simulink model "WarehouseFleetSim"  (R2024b)
settings: Solver=ode4  StartTime=0.0  StopTime=inf  FixedStep=0.02  RelTol=1e-3
StopFcn:
  | try, fleetVisionStep('close'); catch, end; try, phase3('stopped'); catch, end
model workspace (MAT data in the model file):
  HomePose1 = [-20 7.3 0]
  HomePose2 = [-20 3.6 0]
  HomePose3 = [-20 11 0]
  HomePose4 = [-24.5 3.6 0]
  HomePose5 = [-24.5 7.3 0]
  HomePose6 = [-24.5 11 0]
  Zero = 0
  gen3 : robotics.RigidBodyTree (value not decoded)
  qStow = [0; 0; 0.261799387799; 3.14159265359; -2.26892802759; 0; 0.959931088597; 1.57079632679]
undefined symbols (not defined in the file or in its folder): Actor, setupFleetScene, Sim3dSensor, World
libraries: sim3dlib x128, sim3dcameralib x7, robotmobilelib x6, robotsim3dlib x6
(part 1 of 4)
settings Model: Creator=ssuga  LastModifiedBy=ssuga
settings DataIOCC: ReturnWorkspaceOutputs=off

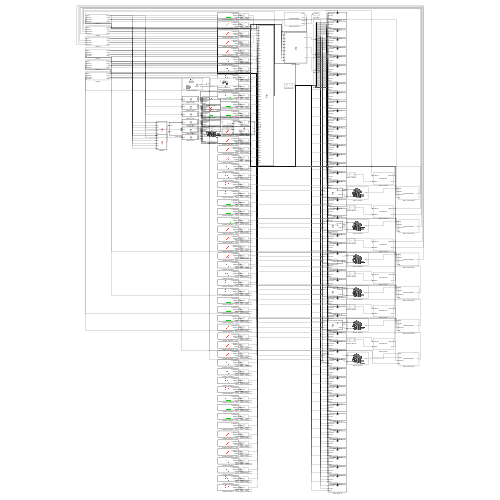
[thumbnail: Simulink's stored preview of the top-level diagram]
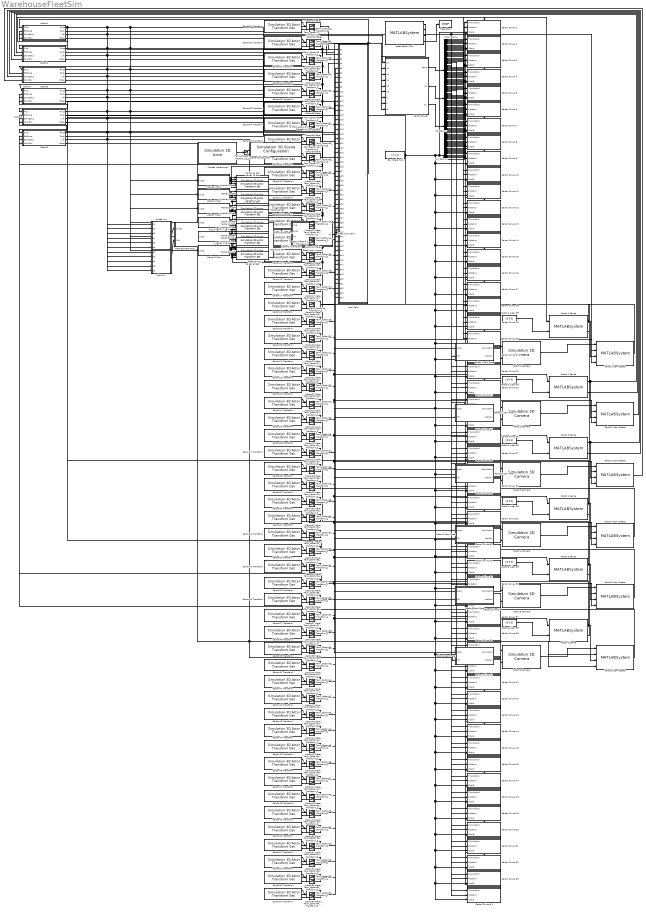
== system WarehouseFleetSim ==
  Box Scale Hold : Constant  Value=[1 1 1]  VectorParams1D=off  OutDataTypeStr=double
  Carton Driver 1 : Subsystem  TreatAsAtomicUnit=on
  Carton Driver 10 : Subsystem  TreatAsAtomicUnit=on
  Carton Driver 11 : Subsystem  TreatAsAtomicUnit=on
  Carton Driver 12 : Subsystem  TreatAsAtomicUnit=on
  Carton Driver 13 : Subsystem  TreatAsAtomicUnit=on
  Carton Driver 14 : Subsystem  TreatAsAtomicUnit=on
  Carton Driver 15 : Subsystem  TreatAsAtomicUnit=on
  Carton Driver 16 : Subsystem  TreatAsAtomicUnit=on
  Carton Driver 17 : Subsystem  TreatAsAtomicUnit=on
  Carton Driver 18 : Subsystem  TreatAsAtomicUnit=on
  Carton Driver 19 : Subsystem  TreatAsAtomicUnit=on
  Carton Driver 2 : Subsystem  TreatAsAtomicUnit=on
  Carton Driver 20 : Subsystem  TreatAsAtomicUnit=on
  Carton Driver 21 : Subsystem  TreatAsAtomicUnit=on
  Carton Driver 22 : Subsystem  TreatAsAtomicUnit=on
  Carton Driver 23 : Subsystem  TreatAsAtomicUnit=on
  Carton Driver 24 : Subsystem  TreatAsAtomicUnit=on
  Carton Driver 25 : Subsystem  TreatAsAtomicUnit=on
  Carton Driver 26 : Subsystem  TreatAsAtomicUnit=on
  Carton Driver 27 : Subsystem  TreatAsAtomicUnit=on
  Carton Driver 28 : Subsystem  TreatAsAtomicUnit=on
  Carton Driver 29 : Subsystem  TreatAsAtomicUnit=on
  Carton Driver 3 : Subsystem  TreatAsAtomicUnit=on
  Carton Driver 30 : Subsystem  TreatAsAtomicUnit=on
  Carton Driver 31 : Subsystem  TreatAsAtomicUnit=on
  Carton Driver 32 : Subsystem  TreatAsAtomicUnit=on
  Carton Driver 33 : Subsystem  TreatAsAtomicUnit=on
  Carton Driver 34 : Subsystem  TreatAsAtomicUnit=on
  Carton Driver 35 : Subsystem  TreatAsAtomicUnit=on
  Carton Driver 36 : Subsystem  TreatAsAtomicUnit=on
  Carton Driver 37 : Subsystem  TreatAsAtomicUnit=on
  Carton Driver 38 : Subsystem  TreatAsAtomicUnit=on
  Carton Driver 39 : Subsystem  TreatAsAtomicUnit=on
  Carton Driver 4 : Subsystem  TreatAsAtomicUnit=on
  Carton Driver 40 : Subsystem  TreatAsAtomicUnit=on
  Carton Driver 41 : Subsystem  TreatAsAtomicUnit=on
  Carton Driver 42 : Subsystem  TreatAsAtomicUnit=on
  Carton Driver 43 : Subsystem  TreatAsAtomicUnit=on
  Carton Driver 44 : Subsystem  TreatAsAtomicUnit=on
  Carton Driver 45 : Subsystem  TreatAsAtomicUnit=on
  Carton Driver 46 : Subsystem  TreatAsAtomicUnit=on
  Carton Driver 47 : Subsystem  TreatAsAtomicUnit=on
  Carton Driver 48 : Subsystem  TreatAsAtomicUnit=on
  Carton Driver 49 : Subsystem  TreatAsAtomicUnit=on
  Carton Driver 5 : Subsystem  TreatAsAtomicUnit=on
  Carton Driver 50 : Subsystem  TreatAsAtomicUnit=on
  Carton Driver 51 : Subsystem  TreatAsAtomicUnit=on
  Carton Driver 52 : Subsystem  TreatAsAtomicUnit=on
  Carton Driver 53 : Subsystem  TreatAsAtomicUnit=on
  Carton Driver 54 : Subsystem  TreatAsAtomicUnit=on
  Carton Driver 6 : Subsystem  TreatAsAtomicUnit=on
  Carton Driver 7 : Subsystem  TreatAsAtomicUnit=on
  Carton Driver 8 : Subsystem  TreatAsAtomicUnit=on
  Carton Driver 9 : Subsystem  TreatAsAtomicUnit=on
  Carton Router : MATLAB Function  TreatAsAtomicUnit=on
  Carton01 Delay : UnitDelay  InitialCondition=[-23.225 -38 1.43]  SampleTime=0.02  HasFrameUpgradeWarning=on
  Carton01 Transform : sim3dlib/Simulation 3D Actor Transform Get  Priority=1  ActorTag=Carton01  NumberOfParts=1  CustNumOfParts=3  Ts=-1  aMode=aMode
  Carton02 Delay : UnitDelay  InitialCondition=[-9.775 -51.4642857142857 0.53]  SampleTime=0.02  HasFrameUpgradeWarning=on
  Carton02 Transform : sim3dlib/Simulation 3D Actor Transform Get  Priority=1  ActorTag=Carton02  NumberOfParts=1  CustNumOfParts=3  Ts=-1  aMode=aMode
  Carton03 Delay : UnitDelay  InitialCondition=[13.225 -46.0555555555556 2.33]  SampleTime=0.02  HasFrameUpgradeWarning=on
  Carton03 Transform : sim3dlib/Simulation 3D Actor Transform Get  Priority=1  ActorTag=Carton03  NumberOfParts=1  CustNumOfParts=3  Ts=-1  aMode=aMode
  Carton04 Delay : UnitDelay  InitialCondition=[11.775 -51.8333333333333 2.33]  SampleTime=0.02  HasFrameUpgradeWarning=on
  Carton04 Transform : sim3dlib/Simulation 3D Actor Transform Get  Priority=1  ActorTag=Carton04  NumberOfParts=1  CustNumOfParts=3  Ts=-1  aMode=aMode
  Carton05 Delay : UnitDelay  InitialCondition=[24.225 -38.4285714285714 0.53]  SampleTime=0.02  HasFrameUpgradeWarning=on
  Carton05 Transform : sim3dlib/Simulation 3D Actor Transform Get  Priority=1  ActorTag=Carton05  NumberOfParts=1  CustNumOfParts=3  Ts=-1  aMode=aMode
  Carton06 Delay : UnitDelay  InitialCondition=[-21.775 -25.1428571428571 1.43]  SampleTime=0.02  HasFrameUpgradeWarning=on
  Carton06 Transform : sim3dlib/Simulation 3D Actor Transform Get  Priority=1  ActorTag=Carton06  NumberOfParts=1  CustNumOfParts=3  Ts=-1  aMode=aMode
  Carton07 Delay : UnitDelay  InitialCondition=[-11.225 -35.1785714285714 1.43]  SampleTime=0.02  HasFrameUpgradeWarning=on
  Carton07 Transform : sim3dlib/Simulation 3D Actor Transform Get  Priority=1  ActorTag=Carton07  NumberOfParts=1  CustNumOfParts=3  Ts=-1  aMode=aMode
  Carton08 Delay : UnitDelay  InitialCondition=[24.225 -22.7142857142857 1.43]  SampleTime=0.02  HasFrameUpgradeWarning=on
  Carton08 Transform : sim3dlib/Simulation 3D Actor Transform Get  Priority=1  ActorTag=Carton08  NumberOfParts=1  CustNumOfParts=3  Ts=-1  aMode=aMode
  Carton09 Delay : UnitDelay  InitialCondition=[-23.225 -50.8571428571429 0.53]  SampleTime=0.02  HasFrameUpgradeWarning=on
  Carton09 Transform : sim3dlib/Simulation 3D Actor Transform Get  Priority=1  ActorTag=Carton09  NumberOfParts=1  CustNumOfParts=3  Ts=-1  aMode=aMode
  Carton10 Delay : UnitDelay  InitialCondition=[-21.775 -39.4285714285714 0.53]  SampleTime=0.02  HasFrameUpgradeWarning=on
  Carton10 Transform : sim3dlib/Simulation 3D Actor Transform Get  Priority=1  ActorTag=Carton10  NumberOfParts=1  CustNumOfParts=3  Ts=-1  aMode=aMode
  Carton11 Delay : UnitDelay  InitialCondition=[24.225 -29.8571428571429 1.43]  SampleTime=0.02  HasFrameUpgradeWarning=on
  Carton11 Transform : sim3dlib/Simulation 3D Actor Transform Get  Priority=1  ActorTag=Carton11  NumberOfParts=1  CustNumOfParts=3  Ts=-1  aMode=aMode
  Carton12 Delay : UnitDelay  InitialCondition=[22.775 -44.1428571428571 1.43]  SampleTime=0.02  HasFrameUpgradeWarning=on
  Carton12 Transform : sim3dlib/Simulation 3D Actor Transform Get  Priority=1  ActorTag=Carton12  NumberOfParts=1  CustNumOfParts=3  Ts=-1  aMode=aMode
  Carton13 Delay : UnitDelay  InitialCondition=[-21.775 -26.5714285714286 1.43]  SampleTime=0.02  HasFrameUpgradeWarning=on
  Carton13 Transform : sim3dlib/Simulation 3D Actor Transform Get  Priority=1  ActorTag=Carton13  NumberOfParts=1  CustNumOfParts=3  Ts=-1  aMode=aMode
  Carton14 Delay : UnitDelay  InitialCondition=[-9.775 -27.3333333333333 1.43]  SampleTime=0.02  HasFrameUpgradeWarning=on
  Carton14 Transform : sim3dlib/Simulation 3D Actor Transform Get  Priority=1  ActorTag=Carton14  NumberOfParts=1  CustNumOfParts=3  Ts=-1  aMode=aMode
  Carton15 Delay : UnitDelay  InitialCondition=[-23.225 -26.5714285714286 2.33]  SampleTime=0.02  HasFrameUpgradeWarning=on
  Carton15 Transform : sim3dlib/Simulation 3D Actor Transform Get  Priority=1  ActorTag=Carton15  NumberOfParts=1  CustNumOfParts=3  Ts=-1  aMode=aMode
  Carton16 Delay : UnitDelay  InitialCondition=[11.775 -50.3888888888889 0.53]  SampleTime=0.02  HasFrameUpgradeWarning=on
  Carton16 Transform : sim3dlib/Simulation 3D Actor Transform Get  Priority=1  ActorTag=Carton16  NumberOfParts=1  CustNumOfParts=3  Ts=-1  aMode=aMode
  Carton17 Delay : UnitDelay  InitialCondition=[24.225 -44.1428571428571 2.33]  SampleTime=0.02  HasFrameUpgradeWarning=on
  Carton17 Transform : sim3dlib/Simulation 3D Actor Transform Get  Priority=1  ActorTag=Carton17  NumberOfParts=1  CustNumOfParts=3  Ts=-1  aMode=aMode
  Carton18 Delay : UnitDelay  InitialCondition=[13.225 -28.8888888888889 0.53]  SampleTime=0.02  HasFrameUpgradeWarning=on
  Carton18 Transform : sim3dlib/Simulation 3D Actor Transform Get  Priority=1  ActorTag=Carton18  NumberOfParts=1  CustNumOfParts=3  Ts=-1  aMode=aMode
  Carton19 Delay : UnitDelay  InitialCondition=[-23.225 -42.2857142857143 1.43]  SampleTime=0.02  HasFrameUpgradeWarning=on
  Carton19 Transform : sim3dlib/Simulation 3D Actor Transform Get  Priority=1  ActorTag=Carton19  NumberOfParts=1  CustNumOfParts=3  Ts=-1  aMode=aMode
  Carton20 Delay : UnitDelay  InitialCondition=[0.275 -37.8928571428571 0.53]  SampleTime=0.02  HasFrameUpgradeWarning=on
  Carton20 Transform : sim3dlib/Simulation 3D Actor Transform Get  Priority=1  ActorTag=Carton20  NumberOfParts=1  CustNumOfParts=3  Ts=-1  aMode=aMode
  Carton21 Delay : UnitDelay  InitialCondition=[0.275 -46.0357142857143 0.53]  SampleTime=0.02  HasFrameUpgradeWarning=on
  Carton21 Transform : sim3dlib/Simulation 3D Actor Transform Get  Priority=1  ActorTag=Carton21  NumberOfParts=1  CustNumOfParts=3  Ts=-1  aMode=aMode
  Carton22 Delay : UnitDelay  InitialCondition=[13.225 -53.2777777777778 0.53]  SampleTime=0.02  HasFrameUpgradeWarning=on
  Carton22 Transform : sim3dlib/Simulation 3D Actor Transform Get  Priority=1  ActorTag=Carton22  NumberOfParts=1  CustNumOfParts=3  Ts=-1  aMode=aMode
  Carton23 Delay : UnitDelay  InitialCondition=[-11.225 -46.0357142857143 2.33]  SampleTime=0.02  HasFrameUpgradeWarning=on
  Carton23 Transform : sim3dlib/Simulation 3D Actor Transform Get  Priority=1  ActorTag=Carton23  NumberOfParts=1  CustNumOfParts=3  Ts=-1  aMode=aMode
  Carton24 Delay : UnitDelay  InitialCondition=[-23.225 -33.7142857142857 0.53]  SampleTime=0.02  HasFrameUpgradeWarning=on
  Carton24 Transform : sim3dlib/Simulation 3D Actor Transform Get  Priority=1  ActorTag=Carton24  NumberOfParts=1  CustNumOfParts=3  Ts=-1  aMode=aMode
  Carton25 Delay : UnitDelay  InitialCondition=[11.775 -30.3333333333333 2.33]  SampleTime=0.02  HasFrameUpgradeWarning=on
  Carton25 Transform : sim3dlib/Simulation 3D Actor Transform Get  Priority=1  ActorTag=Carton25  NumberOfParts=1  CustNumOfParts=3  Ts=-1  aMode=aMode
  Carton26 Delay : UnitDelay  InitialCondition=[-9.775 -25.8888888888889 1.43]  SampleTime=0.02  HasFrameUpgradeWarning=on
  Carton26 Transform : sim3dlib/Simulation 3D Actor Transform Get  Priority=1  ActorTag=Carton26  NumberOfParts=1  CustNumOfParts=3  Ts=-1  aMode=aMode
  Carton27 Delay : UnitDelay  InitialCondition=[11.775 -41.7222222222222 0.53]  SampleTime=0.02  HasFrameUpgradeWarning=on
  Carton27 Transform : sim3dlib/Simulation 3D Actor Transform Get  Priority=1  ActorTag=Carton27  NumberOfParts=1  CustNumOfParts=3  Ts=-1  aMode=aMode
  Carton28 Delay : UnitDelay  InitialCondition=[24.225 -49.8571428571429 0.53]  SampleTime=0.02  HasFrameUpgradeWarning=on
  Carton28 Transform : sim3dlib/Simulation 3D Actor Transform Get  Priority=1  ActorTag=Carton28  NumberOfParts=1  CustNumOfParts=3  Ts=-1  aMode=aMode
  Carton29 Delay : UnitDelay  InitialCondition=[-23.225 -49.4285714285714 2.33]  SampleTime=0.02  HasFrameUpgradeWarning=on
  Carton29 Transform : sim3dlib/Simulation 3D Actor Transform Get  Priority=1  ActorTag=Carton29  NumberOfParts=1  CustNumOfParts=3  Ts=-1  aMode=aMode
  Carton30 Delay : UnitDelay  InitialCondition=[-11.225 -51.4642857142857 2.33]  SampleTime=0.02  HasFrameUpgradeWarning=on
  Carton30 Transform : sim3dlib/Simulation 3D Actor Transform Get  Priority=1  ActorTag=Carton30  NumberOfParts=1  CustNumOfParts=3  Ts=-1  aMode=aMode
  Carton31 Delay : UnitDelay  InitialCondition=[-11 -3.775 0.53]  SampleTime=0.02  HasFrameUpgradeWarning=on
  Carton31 Transform : sim3dlib/Simulation 3D Actor Transform Get  Priority=1  ActorTag=Carton31  NumberOfParts=1  CustNumOfParts=3  Ts=-1  aMode=aMode
  Carton32 Delay : UnitDelay  InitialCondition=[-8.5 -3.775 0.53]  SampleTime=0.02  HasFrameUpgradeWarning=on
  Carton32 Transform : sim3dlib/Simulation 3D Actor Transform Get  Priority=1  ActorTag=Carton32  NumberOfParts=1  CustNumOfParts=3  Ts=-1  aMode=aMode
  Carton33 Delay : UnitDelay  InitialCondition=[-6 -3.775 0.53]  SampleTime=0.02  HasFrameUpgradeWarning=on
  Carton33 Transform : sim3dlib/Simulation 3D Actor Transform Get  Priority=1  ActorTag=Carton33  NumberOfParts=1  CustNumOfParts=3  Ts=-1  aMode=aMode
  Carton34 Delay : UnitDelay  InitialCondition=[-3.5 -3.775 0.53]  SampleTime=0.02  HasFrameUpgradeWarning=on
  Carton34 Transform : sim3dlib/Simulation 3D Actor Transform Get  Priority=1  ActorTag=Carton34  NumberOfParts=1  CustNumOfParts=3  Ts=-1  aMode=aMode
  Carton35 Delay : UnitDelay  InitialCondition=[1.5 -3.775 0.53]  SampleTime=0.02  HasFrameUpgradeWarning=on
  Carton35 Transform : sim3dlib/Simulation 3D Actor Transform Get  Priority=1  ActorTag=Carton35  NumberOfParts=1  CustNumOfParts=3  Ts=-1  aMode=aMode
  Carton36 Delay : UnitDelay  InitialCondition=[4 -3.775 0.53]  SampleTime=0.02  HasFrameUpgradeWarning=on
  Carton36 Transform : sim3dlib/Simulation 3D Actor Transform Get  Priority=1  ActorTag=Carton36  NumberOfParts=1  CustNumOfParts=3  Ts=-1  aMode=aMode
  Carton37 Delay : UnitDelay  InitialCondition=[6.5 -3.775 0.53]  SampleTime=0.02  HasFrameUpgradeWarning=on
  Carton37 Transform : sim3dlib/Simulation 3D Actor Transform Get  Priority=1  ActorTag=Carton37  NumberOfParts=1  CustNumOfParts=3  Ts=-1  aMode=aMode
  Carton38 Delay : UnitDelay  InitialCondition=[9 -3.775 0.53]  SampleTime=0.02  HasFrameUpgradeWarning=on
  Carton38 Transform : sim3dlib/Simulation 3D Actor Transform Get  Priority=1  ActorTag=Carton38  NumberOfParts=1  CustNumOfParts=3  Ts=-1  aMode=aMode
  Carton39 Delay : UnitDelay  InitialCondition=[11.5 -3.775 0.53]  SampleTime=0.02  HasFrameUpgradeWarning=on
  Carton39 Transform : sim3dlib/Simulation 3D Actor Transform Get  Priority=1  ActorTag=Carton39  NumberOfParts=1  CustNumOfParts=3  Ts=-1  aMode=aMode
  Carton40 Delay : UnitDelay  InitialCondition=[15.5 -3.775 0.53]  SampleTime=0.02  HasFrameUpgradeWarning=on
  Carton40 Transform : sim3dlib/Simulation 3D Actor Transform Get  Priority=1  ActorTag=Carton40  NumberOfParts=1  CustNumOfParts=3  Ts=-1  aMode=aMode
  Carton41 Delay : UnitDelay  InitialCondition=[-3 -39 -3]  SampleTime=0.02  HasFrameUpgradeWarning=on
  Carton41 Transform : sim3dlib/Simulation 3D Actor Transform Get  Priority=1  ActorTag=Carton41  NumberOfParts=1  CustNumOfParts=3  Ts=-1  aMode=aMode
  Carton42 Delay : UnitDelay  InitialCondition=[-2.1 -39 -3]  SampleTime=0.02  HasFrameUpgradeWarning=on
  Carton42 Transform : sim3dlib/Simulation 3D Actor Transform Get  Priority=1  ActorTag=Carton42  NumberOfParts=1  CustNumOfParts=3  Ts=-1  aMode=aMode
  Carton43 Delay : UnitDelay  InitialCondition=[-1.2 -39 -3]  SampleTime=0.02  HasFrameUpgradeWarning=on
  Carton43 Transform : sim3dlib/Simulation 3D Actor Transform Get  Priority=1  ActorTag=Carton43  NumberOfParts=1  CustNumOfParts=3  Ts=-1  aMode=aMode
  Carton44 Delay : UnitDelay  InitialCondition=[-0.3 -39 -3]  SampleTime=0.02  HasFrameUpgradeWarning=on
  Carton44 Transform : sim3dlib/Simulation 3D Actor Transform Get  Priority=1  ActorTag=Carton44  NumberOfParts=1  CustNumOfParts=3  Ts=-1  aMode=aMode
  Carton45 Delay : UnitDelay  InitialCondition=[-3 -39.9 -3]  SampleTime=0.02  HasFrameUpgradeWarning=on
  Carton45 Transform : sim3dlib/Simulation 3D Actor Transform Get  Priority=1  ActorTag=Carton45  NumberOfParts=1  CustNumOfParts=3  Ts=-1  aMode=aMode
  Carton46 Delay : UnitDelay  InitialCondition=[-2.1 -39.9 -3]  SampleTime=0.02  HasFrameUpgradeWarning=on
  Carton46 Transform : sim3dlib/Simulation 3D Actor Transform Get  Priority=1  ActorTag=Carton46  NumberOfParts=1  CustNumOfParts=3  Ts=-1  aMode=aMode
  Carton47 Delay : UnitDelay  InitialCondition=[-1.2 -39.9 -3]  SampleTime=0.02  HasFrameUpgradeWarning=on
  Carton47 Transform : sim3dlib/Simulation 3D Actor Transform Get  Priority=1  ActorTag=Carton47  NumberOfParts=1  CustNumOfParts=3  Ts=-1  aMode=aMode
  Carton48 Delay : UnitDelay  InitialCondition=[-0.3 -39.9 -3]  SampleTime=0.02  HasFrameUpgradeWarning=on
  Carton48 Transform : sim3dlib/Simulation 3D Actor Transform Get  Priority=1  ActorTag=Carton48  NumberOfParts=1  CustNumOfParts=3  Ts=-1  aMode=aMode
  Carton49 Delay : UnitDelay  InitialCondition=[-3 -40.8 -3]  SampleTime=0.02  HasFrameUpgradeWarning=on
  Carton49 Transform : sim3dlib/Simulation 3D Actor Transform Get  Priority=1  ActorTag=Carton49  NumberOfParts=1  CustNumOfParts=3  Ts=-1  aMode=aMode
  Carton50 Delay : UnitDelay  InitialCondition=[-2.1 -40.8 -3]  SampleTime=0.02  HasFrameUpgradeWarning=on
  Carton50 Transform : sim3dlib/Simulation 3D Actor Transform Get  Priority=1  ActorTag=Carton50  NumberOfParts=1  CustNumOfParts=3  Ts=-1  aMode=aMode
  Carton51 Delay : UnitDelay  InitialCondition=[-1.2 -40.8 -3]  SampleTime=0.02  HasFrameUpgradeWarning=on
  Carton51 Transform : sim3dlib/Simulation 3D Actor Transform Get  Priority=1  ActorTag=Carton51  NumberOfParts=1  CustNumOfParts=3  Ts=-1  aMode=aMode
  Carton52 Delay : UnitDelay  InitialCondition=[-0.3 -40.8 -3]  SampleTime=0.02  HasFrameUpgradeWarning=on
  Carton52 Transform : sim3dlib/Simulation 3D Actor Transform Get  Priority=1  ActorTag=Carton52  NumberOfParts=1  CustNumOfParts=3  Ts=-1  aMode=aMode
  Carton53 Delay : UnitDelay  InitialCondition=[-3 -41.7 -3]  SampleTime=0.02  HasFrameUpgradeWarning=on
  Carton53 Transform : sim3dlib/Simulation 3D Actor Transform Get  Priority=1  ActorTag=Carton53  NumberOfParts=1  CustNumOfParts=3  Ts=-1  aMode=aMode
  Carton54 Delay : UnitDelay  InitialCondition=[-2.1 -41.7 -3]  SampleTime=0.02  HasFrameUpgradeWarning=on
  Carton54 Transform : sim3dlib/Simulation 3D Actor Transform Get  Priority=1  ActorTag=Carton54  NumberOfParts=1  CustNumOfParts=3  Ts=-1  aMode=aMode
  Drv Demux : Demux  Outputs=54
  Fleet Camera : sim3dcameralib/Simulation 3D Camera  Priority=1  sensorTag=Sim3dSensor�  sensorId=17  sensorName=Sim3dSensor�  vehTagList={'<empty>';'Ro1Kinova';'Ro2Kinova';'Ro3Kinova';'Ro4Kinova';'Ro5Kinova';'Ro6Kinova';'Scene Origin';'WarehouseRoot'}  vehTag=Scene Origin  mountLoc=Origin  offsetFlag=on  tmountOffset=[0, 0, 0]  extTmount=on  rmountOffset=[0, 0, 0]  extRmount=on  FocalLength=[300 300]  OpticalCenter=[320 240]  ImageSize=[480 640]  RadialDistortion=[0, 0]  TangentialDistortion=[0, 0]  SensorSkew=0  DepthOutportEnabled=off  SemanticOutportEnabled=off  TransformOutportEnabled=off  SampleTime=0.1  mountPoint=[0 0 0]  mountOrientation=[0 0 0]  aMode=aMode  ID=17
  Fleet Camera Pose : MATLAB Function  TreatAsAtomicUnit=on
  Fleet Carton Cmd : MATLABSystem  System=Phase3FleetBlock  NumCartons=54  SampleTime=0.02  SimulateUsing=Interpreted execution
      mask Type: Phase3FleetBlock
      mask Display:
      | disp('Phase3FleetBlock');
      | port_label('output',1,'cmd');
      | port_label('output',2,'rotc');
      | port_label('output',3,'act');
      | port_label('output',4,'stop');
  Fleet Stop : Stop
  Fleet Vision End : Terminator
  Fleet Vision Viewer : MATLAB Function  TreatAsAtomicUnit=on
  Lifts Mux : MATLAB Function  TreatAsAtomicUnit=on
  Marker 1 Calc : MATLAB Function  TreatAsAtomicUnit=on
  Marker 1a Set : sim3dlib/Simulation 3D Actor Transform Set  Priority=1  ActorTag=RobotMarker1_1  NumberOfParts=1  CustNumOfParts=3  Translation=[0 0 0]  Rotation=[0 0 0]  Scale=[1 1 1]  Ts=-1  aMode=aMode
  Marker 1b Set : sim3dlib/Simulation 3D Actor Transform Set  Priority=1  ActorTag=RobotMarker1_2  NumberOfParts=1  CustNumOfParts=3  Translation=[0 0 0]  Rotation=[0 0 0]  Scale=[1 1 1]  Ts=-1  aMode=aMode
  Marker 1c Set : sim3dlib/Simulation 3D Actor Transform Set  Priority=1  ActorTag=RobotMarker1_3  NumberOfParts=1  CustNumOfParts=3  Translation=[0 0 0]  Rotation=[0 0 0]  Scale=[1 1 1]  Ts=-1  aMode=aMode
  Marker 2 Calc : MATLAB Function  TreatAsAtomicUnit=on
  Marker 2a Set : sim3dlib/Simulation 3D Actor Transform Set  Priority=1  ActorTag=RobotMarker2_1  NumberOfParts=1  CustNumOfParts=3  Translation=[0 0 0]  Rotation=[0 0 0]  Scale=[1 1 1]  Ts=-1  aMode=aMode
  Marker 2b Set : sim3dlib/Simulation 3D Actor Transform Set  Priority=1  ActorTag=RobotMarker2_2  NumberOfParts=1  CustNumOfParts=3  Translation=[0 0 0]  Rotation=[0 0 0]  Scale=[1 1 1]  Ts=-1  aMode=aMode
  Marker 2c Set : sim3dlib/Simulation 3D Actor Transform Set  Priority=1  ActorTag=RobotMarker2_3  NumberOfParts=1  CustNumOfParts=3  Translation=[0 0 0]  Rotation=[0 0 0]  Scale=[1 1 1]  Ts=-1  aMode=aMode
  Marker 3 Calc : MATLAB Function  TreatAsAtomicUnit=on
  Marker 3a Set : sim3dlib/Simulation 3D Actor Transform Set  Priority=1  ActorTag=RobotMarker3_1  NumberOfParts=1  CustNumOfParts=3  Translation=[0 0 0]  Rotation=[0 0 0]  Scale=[1 1 1]  Ts=-1  aMode=aMode
  Marker 3b Set : sim3dlib/Simulation 3D Actor Transform Set  Priority=1  ActorTag=RobotMarker3_2  NumberOfParts=1  CustNumOfParts=3  Translation=[0 0 0]  Rotation=[0 0 0]  Scale=[1 1 1]  Ts=-1  aMode=aMode
  Marker 3c Set : sim3dlib/Simulation 3D Actor Transform Set  Priority=1  ActorTag=RobotMarker3_3  NumberOfParts=1  CustNumOfParts=3  Translation=[0 0 0]  Rotation=[0 0 0]  Scale=[1 1 1]  Ts=-1  aMode=aMode
  Marker 4 Calc : MATLAB Function  TreatAsAtomicUnit=on
  Marker 4a Set : sim3dlib/Simulation 3D Actor Transform Set  Priority=1  ActorTag=RobotMarker4_1  NumberOfParts=1  CustNumOfParts=3  Translation=[0 0 0]  Rotation=[0 0 0]  Scale=[1 1 1]  Ts=-1  aMode=aMode
  Marker 4b Set : sim3dlib/Simulation 3D Actor Transform Set  Priority=1  ActorTag=RobotMarker4_2  NumberOfParts=1  CustNumOfParts=3  Translation=[0 0 0]  Rotation=[0 0 0]  Scale=[1 1 1]  Ts=-1  aMode=aMode
  Marker 4c Set : sim3dlib/Simulation 3D Actor Transform Set  Priority=1  ActorTag=RobotMarker4_3  NumberOfParts=1  CustNumOfParts=3  Translation=[0 0 0]  Rotation=[0 0 0]  Scale=[1 1 1]  Ts=-1  aMode=aMode
  Marker 5 Calc : MATLAB Function  TreatAsAtomicUnit=on
  Marker 5a Set : sim3dlib/Simulation 3D Actor Transform Set  Priority=1  ActorTag=RobotMarker5_1  NumberOfParts=1  CustNumOfParts=3  Translation=[0 0 0]  Rotation=[0 0 0]  Scale=[1 1 1]  Ts=-1  aMode=aMode
  Marker 5b Set : sim3dlib/Simulation 3D Actor Transform Set  Priority=1  ActorTag=RobotMarker5_2  NumberOfParts=1  CustNumOfParts=3  Translation=[0 0 0]  Rotation=[0 0 0]  Scale=[1 1 1]  Ts=-1  aMode=aMode
  Marker 5c Set : sim3dlib/Simulation 3D Actor Transform Set  Priority=1  ActorTag=RobotMarker5_3  NumberOfParts=1  CustNumOfParts=3  Translation=[0 0 0]  Rotation=[0 0 0]  Scale=[1 1 1]  Ts=-1  aMode=aMode
  Marker 6 Calc : MATLAB Function  TreatAsAtomicUnit=on
  Marker 6a Set : sim3dlib/Simulation 3D Actor Transform Set  Priority=1  ActorTag=RobotMarker6_1  NumberOfParts=1  CustNumOfParts=3  Translation=[0 0 0]  Rotation=[0 0 0]  Scale=[1 1 1]  Ts=-1  aMode=aMode
  Marker 6b Set : sim3dlib/Simulation 3D Actor Transform Set  Priority=1  ActorTag=RobotMarker6_2  NumberOfParts=1  CustNumOfParts=3  Translation=[0 0 0]  Rotation=[0 0 0]  Scale=[1 1 1]  Ts=-1  aMode=aMode
  Marker 6c Set : sim3dlib/Simulation 3D Actor Transform Set  Priority=1  ActorTag=RobotMarker6_3  NumberOfParts=1  CustNumOfParts=3  Translation=[0 0 0]  Rotation=[0 0 0]  Scale=[1 1 1]  Ts=-1  aMode=aMode
  Phase3 Warehouse : sim3dlib/Simulation 3D Actor  Priority=1  ActorName=WarehouseRoot  ParentName=Scene Origin  Operation=Create at setup  InitScriptText=setupFleetScene(Actor,World);  SampleTime=-1  Translation=[0 0 0]  Rotation=[0 0 0]  Scale=[1 1 1]  aMode=aMode  ActorTag=WarehouseRoot  ActorType=Sim3dActor  ID=C
  Pool Pack : MATLAB Function  TreatAsAtomicUnit=on
  Poses Mux : MATLAB Function  TreatAsAtomicUnit=on
  Robot 1 : Subsystem
  Robot 1 Cam Detect : MATLABSystem  System=Phase3CamDetect  RobotId=1  SimulateUsing=Interpreted execution
      mask Type: Phase3CamDetect
      mask Display:
      | disp('Phase3CamDetect');
      | port_label('input',1,'img');
      | port_label('input',2,'state');
      | port_label('input',3,'estPose');
      | port_label('input',4,'lift');
      | port_label('output',1,'out');
  Robot 1 Cam Pose : MATLAB Function  TreatAsAtomicUnit=on
  Robot 1 Camera : sim3dcameralib/Simulation 3D Camera  Priority=1  sensorTag=Sim3dSensor�  sensorId=11  sensorName=Sim3dSensor�  vehTagList={'<empty>';'Ro1Kinova';'Ro2Kinova';'Ro3Kinova';'Ro4Kinova';'Ro5Kinova';'Ro6Kinova';'Scene Origin';'WarehouseRoot'}  vehTag=Scene Origin  mountLoc=Origin  offsetFlag=on  tmountOffset=[0, 0, 0]  extTmount=on  rmountOffset=[0, 0, 0]  extRmount=on  FocalLength=[300 300]  OpticalCenter=[320 240]  ImageSize=[480 640]  RadialDistortion=[0, 0]  TangentialDistortion=[0, 0]  SensorSkew=0  DepthOutportEnabled=off  SemanticOutportEnabled=off  TransformOutportEnabled=off  SampleTime=0.4  mountPoint=[0 0 0]  mountOrientation=[0 0 0]  aMode=aMode  ID=11
  Robot 1 Lidar Off : Constant  Value=[0 0 0]  VectorParams1D=off  OutDataTypeStr=double
  Robot 1 Sense : MATLABSystem  System=Phase3Sense  RobotId=1  SimulateUsing=Interpreted execution
      mask Type: Phase3Sense
      mask Display:
      | disp('Phase3Sense');
      | port_label('input',1,'truePose');
      | port_label('input',2,'lidarPC');
      | port_label('output',1,'estPose');
      | port_label('output',2,'bus');
  Robot 2 : Subsystem
  Robot 2 Cam Detect : MATLABSystem  System=Phase3CamDetect  RobotId=2  SimulateUsing=Interpreted execution
      mask Type: Phase3CamDetect
      mask Display:
      | disp('Phase3CamDetect');
      | port_label('input',1,'img');
      | port_label('input',2,'state');
      | port_label('input',3,'estPose');
      | port_label('input',4,'lift');
      | port_label('output',1,'out');
  Robot 2 Cam Pose : MATLAB Function  TreatAsAtomicUnit=on
  Robot 2 Camera : sim3dcameralib/Simulation 3D Camera  Priority=1  sensorTag=Sim3dSensor�  sensorId=12  sensorName=Sim3dSensor�  vehTagList={'<empty>';'Ro1Kinova';'Ro2Kinova';'Ro3Kinova';'Ro4Kinova';'Ro5Kinova';'Ro6Kinova';'Scene Origin';'WarehouseRoot'}  vehTag=Scene Origin  mountLoc=Origin  offsetFlag=on  tmountOffset=[0, 0, 0]  extTmount=on  rmountOffset=[0, 0, 0]  extRmount=on  FocalLength=[300 300]  OpticalCenter=[320 240]  ImageSize=[480 640]  RadialDistortion=[0, 0]  TangentialDistortion=[0, 0]  SensorSkew=0  DepthOutportEnabled=off  SemanticOutportEnabled=off  TransformOutportEnabled=off  SampleTime=0.4  mountPoint=[0 0 0]  mountOrientation=[0 0 0]  aMode=aMode  ID=12
  Robot 2 Lidar Off : Constant  Value=[0 0 0]  VectorParams1D=off  OutDataTypeStr=double
  Robot 2 Sense : MATLABSystem  System=Phase3Sense  RobotId=2  SimulateUsing=Interpreted execution
      mask Type: Phase3Sense
      mask Display:
      | disp('Phase3Sense');
      | port_label('input',1,'truePose');
      | port_label('input',2,'lidarPC');
      | port_label('output',1,'estPose');
      | port_label('output',2,'bus');
  Robot 3 : Subsystem
  Robot 3 Cam Detect : MATLABSystem  System=Phase3CamDetect  RobotId=3  SimulateUsing=Interpreted execution
      mask Type: Phase3CamDetect
      mask Display:
      | disp('Phase3CamDetect');
      | port_label('input',1,'img');
      | port_label('input',2,'state');
      | port_label('input',3,'estPose');
      | port_label('input',4,'lift');
      | port_label('output',1,'out');
  Robot 3 Cam Pose : MATLAB Function  TreatAsAtomicUnit=on
  Robot 3 Camera : sim3dcameralib/Simulation 3D Camera  Priority=1  sensorTag=Sim3dSensor  sensorId=13  sensorName=Sim3dSensor  vehTagList={'<empty>';'Ro1Kinova';'Ro2Kinova';'Ro3Kinova';'Ro4Kinova';'Ro5Kinova';'Ro6Kinova';'Scene Origin';'WarehouseRoot'}  vehTag=Scene Origin  mountLoc=Origin  offsetFlag=on  tmountOffset=[0, 0, 0]  extTmount=on  rmountOffset=[0, 0, 0]  extRmount=on  FocalLength=[300 300]  OpticalCenter=[320 240]  ImageSize=[480 640]  RadialDistortion=[0, 0]  TangentialDistortion=[0, 0]  SensorSkew=0  DepthOutportEnabled=off  SemanticOutportEnabled=off  TransformOutportEnabled=off  SampleTime=0.4  mountPoint=[0 0 0]  mountOrientation=[0 0 0]  aMode=aMode  ID=13
  Robot 3 Lidar Off : Constant  Value=[0 0 0]  VectorParams1D=off  OutDataTypeStr=double
  Robot 3 Sense : MATLABSystem  System=Phase3Sense  RobotId=3  SimulateUsing=Interpreted execution
      mask Type: Phase3Sense
      mask Display:
      | disp('Phase3Sense');
      | port_label('input',1,'truePose');
      | port_label('input',2,'lidarPC');
      | port_label('output',1,'estPose');
      | port_label('output',2,'bus');
  Robot 4 : Subsystem
  Robot 4 Cam Detect : MATLABSystem  System=Phase3CamDetect  RobotId=4  SimulateUsing=Interpreted execution
      mask Type: Phase3CamDetect
      mask Display:
      | disp('Phase3CamDetect');
      | port_label('input',1,'img');
      | port_label('input',2,'state');
      | port_label('input',3,'estPose');
      | port_label('input',4,'lift');
      | port_label('output',1,'out');
  Robot 4 Cam Pose : MATLAB Function  TreatAsAtomicUnit=on
  Robot 4 Camera : sim3dcameralib/Simulation 3D Camera  Priority=1  sensorTag=Sim3dSensor�  sensorId=14  sensorName=Sim3dSensor�  vehTagList={'<empty>';'Ro1Kinova';'Ro2Kinova';'Ro3Kinova';'Ro4Kinova';'Ro5Kinova';'Ro6Kinova';'Scene Origin';'WarehouseRoot'}  vehTag=Scene Origin  mountLoc=Origin  offsetFlag=on  tmountOffset=[0, 0, 0]  extTmount=on  rmountOffset=[0, 0, 0]  extRmount=on  FocalLength=[300 300]  OpticalCenter=[320 240]  ImageSize=[480 640]  RadialDistortion=[0, 0]  TangentialDistortion=[0, 0]  SensorSkew=0  DepthOutportEnabled=off  SemanticOutportEnabled=off  TransformOutportEnabled=off  SampleTime=0.4  mountPoint=[0 0 0]  mountOrientation=[0 0 0]  aMode=aMode  ID=14
  Robot 4 Lidar Off : Constant  Value=[0 0 0]  VectorParams1D=off  OutDataTypeStr=double
  Robot 4 Sense : MATLABSystem  System=Phase3Sense  RobotId=4  SimulateUsing=Interpreted execution
      mask Type: Phase3Sense
      mask Display:
      | disp('Phase3Sense');
      | port_label('input',1,'truePose');
      | port_label('input',2,'lidarPC');
      | port_label('output',1,'estPose');
      | port_label('output',2,'bus');
  Robot 5 : Subsystem
  Robot 5 Cam Detect : MATLABSystem  System=Phase3CamDetect  RobotId=5  SimulateUsing=Interpreted execution
      mask Type: Phase3CamDetect
      mask Display:
      | disp('Phase3CamDetect');
      | port_label('input',1,'img');
      | port_label('input',2,'state');
      | port_label('input',3,'estPose');
      | port_label('input',4,'lift');
      | port_label('output',1,'out');
  Robot 5 Cam Pose : MATLAB Function  TreatAsAtomicUnit=on
  Robot 5 Camera : sim3dcameralib/Simulation 3D Camera  Priority=1  sensorTag=Sim3dSensor�  sensorId=15  sensorName=Sim3dSensor�  vehTagList={'<empty>';'Ro1Kinova';'Ro2Kinova';'Ro3Kinova';'Ro4Kinova';'Ro5Kinova';'Ro6Kinova';'Scene Origin';'WarehouseRoot'}  vehTag=Scene Origin  mountLoc=Origin  offsetFlag=on  tmountOffset=[0, 0, 0]  extTmount=on  rmountOffset=[0, 0, 0]  extRmount=on  FocalLength=[300 300]  OpticalCenter=[320 240]  ImageSize=[480 640]  RadialDistortion=[0, 0]  TangentialDistortion=[0, 0]  SensorSkew=0  DepthOutportEnabled=off  SemanticOutportEnabled=off  TransformOutportEnabled=off  SampleTime=0.4  mountPoint=[0 0 0]  mountOrientation=[0 0 0]  aMode=aMode  ID=15
  Robot 5 Lidar Off : Constant  Value=[0 0 0]  VectorParams1D=off  OutDataTypeStr=double
  Robot 5 Sense : MATLABSystem  System=Phase3Sense  RobotId=5  SimulateUsing=Interpreted execution
      mask Type: Phase3Sense
      mask Display:
      | disp('Phase3Sense');
      | port_label('input',1,'truePose');
      | port_label('input',2,'lidarPC');
      | port_label('output',1,'estPose');
      | port_label('output',2,'bus');
  Robot 6 : Subsystem
  Robot 6 Cam Detect : MATLABSystem  System=Phase3CamDetect  RobotId=6  SimulateUsing=Interpreted execution
      mask Type: Phase3CamDetect
      mask Display:
      | disp('Phase3CamDetect');
      | port_label('input',1,'img');
      | port_label('input',2,'state');
      | port_label('input',3,'estPose');
      | port_label('input',4,'lift');
      | port_label('output',1,'out');
  Robot 6 Cam Pose : MATLAB Function  TreatAsAtomicUnit=on
  Robot 6 Camera : sim3dcameralib/Simulation 3D Camera  Priority=1  sensorTag=Sim3dSensor�  sensorId=16  sensorName=Sim3dSensor�  vehTagList={'<empty>';'Ro1Kinova';'Ro2Kinova';'Ro3Kinova';'Ro4Kinova';'Ro5Kinova';'Ro6Kinova';'Scene Origin';'WarehouseRoot'}  vehTag=Scene Origin  mountLoc=Origin  offsetFlag=on  tmountOffset=[0, 0, 0]  extTmount=on  rmountOffset=[0, 0, 0]  extRmount=on  FocalLength=[300 300]  OpticalCenter=[320 240]  ImageSize=[480 640]  RadialDistortion=[0, 0]  TangentialDistortion=[0, 0]  SensorSkew=0  DepthOutportEnabled=off  SemanticOutportEnabled=off  TransformOutportEnabled=off  SampleTime=0.4  mountPoint=[0 0 0]  mountOrientation=[0 0 0]  aMode=aMode  ID=16
  Robot 6 Lidar Off : Constant  Value=[0 0 0]  VectorParams1D=off  OutDataTypeStr=double
  Robot 6 Sense : MATLABSystem  System=Phase3Sense  RobotId=6  SimulateUsing=Interpreted execution
      mask Type: Phase3Sense
      mask Display:
      | disp('Phase3Sense');
      | port_label('input',1,'truePose');
      | port_label('input',2,'lidarPC');
      | port_label('output',1,'estPose');
      | port_label('output',2,'bus');
  Rot Demux : Demux  Outputs=[3 3 3 3 3 3 3 3 3 3 3 3 3 3 3 3 3 3 3 3 3 3 3 3 3 3 3 3 3 3 3 3 3 3 3 3 3 3 3 3 3 3 3 3 3 3 3 3 3 3 3 3 3 3]
  Scene Configuration : sim3dlib/Simulation 3D Scene Configuration  Priority=0  ProjectFormat=Default Scenes  SceneDesc=Empty scene  ProjectName=C:\Program Files\MATLAB\R2024b\toolbox\shared\sim3d_projects\automotive_project_windows\UE\WindowsNoEditor\VehicleSimulation.exe  ScenePath=/Game/Maps/HwStrght  EnableOpenDRIVE=off  vehTagList={'Scene Origin'}  vehTag=Scene Origin  FreeCameraInitialTranslation=[0, 0, 0]  FreeCameraDefaultInitialTranslation=[-6, 0, 2]  FreeCameraInitialRotation=[0, 0, 0]  FreeCameraDefaultInitialRotation=[0, -15, 0]  OpVisEn=off  Ts=0.02  EnableWindow=on  EnableRemoteAccess=off  EnableWeather=off  SunAzimuth=90  SunAltitude=40.0  EnableGeospatialSun=off  Latitude=0  Longitude=0  Date=2023-01-01  Time=10:30:00  GeoTimeZone=-5.0  SunDaylightSaving=off  wind=1  clouds=10  EnableVolumetricClouds=off  CloudCoverage=0  CloudAltitude=6  fog=0  rain=0  RaindropsEffect=off  SnowDensity=0  EnableGeospatial=off  UseTrueOrigin=off  OriginHeight=200  OriginLatitude=40.744652  OriginLongitude=-73.988864  MapStyle=Aerial  AdditionalAssetIDs=[]  UseAdvancedSunSky=off  SolarTime=11  TimeZone=-5  Day=21  Month=9  Year=2022  UseDaylightSavingTime=on  DSTStartDay=10  DSTStartMonth=3  DSTEndDay=3  DSTEndMonth=11  DSTSwitchHour=2  sensorTag=MainCamera1  sensorId=1  sensorName=MainCamera1  mountLoc=Origin  offsetFlag=off  tmountOffset=[0, 0, 0]  rmountOffset=[0, 0, 0]  HorizontalResolution=1280  VerticalResolution=720  HorizontalFOV=60  mountPoint=[0 0 0]  mountOrientation=[0 0 0]  aMode=aMode  ID=1  GeoTrigger=Inactive
  Term_Carton01_Transform_2 : Terminator
  Term_Carton01_Transform_3 : Terminator
  Term_Carton02_Transform_2 : Terminator
  Term_Carton02_Transform_3 : Terminator
  Term_Carton03_Transform_2 : Terminator
  Term_Carton03_Transform_3 : Terminator
  Term_Carton04_Transform_2 : Terminator
  Term_Carton04_Transform_3 : Terminator
  Term_Carton05_Transform_2 : Terminator
  Term_Carton05_Transform_3 : Terminator
  Term_Carton06_Transform_2 : Terminator
  Term_Carton06_Transform_3 : Terminator
  Term_Carton07_Transform_2 : Terminator
  Term_Carton07_Transform_3 : Terminator
  Term_Carton08_Transform_2 : Terminator
  Term_Carton08_Transform_3 : Terminator
  Term_Carton09_Transform_2 : Terminator
  Term_Carton09_Transform_3 : Terminator
  Term_Carton10_Transform_2 : Terminator
  Term_Carton10_Transform_3 : Terminator
  Term_Carton11_Transform_2 : Terminator
  Term_Carton11_Transform_3 : Terminator
  Term_Carton12_Transform_2 : Terminator
  Term_Carton12_Transform_3 : Terminator
  Term_Carton13_Transform_2 : Terminator
  Term_Carton13_Transform_3 : Terminator
  Term_Carton14_Transform_2 : Terminator
  Term_Carton14_Transform_3 : Terminator
  Term_Carton15_Transform_2 : Terminator
  Term_Carton15_Transform_3 : Terminator
  Term_Carton16_Transform_2 : Terminator
  Term_Carton16_Transform_3 : Terminator
  Term_Carton17_Transform_2 : Terminator
  Term_Carton17_Transform_3 : Terminator
  Term_Carton18_Transform_2 : Terminator
  Term_Carton18_Transform_3 : Terminator
  Term_Carton19_Transform_2 : Terminator
  Term_Carton19_Transform_3 : Terminator
  Term_Carton20_Transform_2 : Terminator
  Term_Carton20_Transform_3 : Terminator
  Term_Carton21_Transform_2 : Terminator
  Term_Carton21_Transform_3 : Terminator
  Term_Carton22_Transform_2 : Terminator
  Term_Carton22_Transform_3 : Terminator
  Term_Carton23_Transform_2 : Terminator
  Term_Carton23_Transform_3 : Terminator
  Term_Carton24_Transform_2 : Terminator
  Term_Carton24_Transform_3 : Terminator
  Term_Carton25_Transform_2 : Terminator
  Term_Carton25_Transform_3 : Terminator
  Term_Carton26_Transform_2 : Terminator
  Term_Carton26_Transform_3 : Terminator
  Term_Carton27_Transform_2 : Terminator
  Term_Carton27_Transform_3 : Terminator
  Term_Carton28_Transform_2 : Terminator
  Term_Carton28_Transform_3 : Terminator
  Term_Carton29_Transform_2 : Terminator
  Term_Carton29_Transform_3 : Terminator
  Term_Carton30_Transform_2 : Terminator
  Term_Carton30_Transform_3 : Terminator
  Term_Carton31_Transform_2 : Terminator
  Term_Carton31_Transform_3 : Terminator
  Term_Carton32_Transform_2 : Terminator
  Term_Carton32_Transform_3 : Terminator
  Term_Carton33_Transform_2 : Terminator
  Term_Carton33_Transform_3 : Terminator
  Term_Carton34_Transform_2 : Terminator
  Term_Carton34_Transform_3 : Terminator
  Term_Carton35_Transform_2 : Terminator
  Term_Carton35_Transform_3 : Terminator
  Term_Carton36_Transform_2 : Terminator
  Term_Carton36_Transform_3 : Terminator
  Term_Carton37_Transform_2 : Terminator
  Term_Carton37_Transform_3 : Terminator
  Term_Carton38_Transform_2 : Terminator
  Term_Carton38_Transform_3 : Terminator
  Term_Carton39_Transform_2 : Terminator
  Term_Carton39_Transform_3 : Terminator
  Term_Carton40_Transform_2 : Terminator
  Term_Carton40_Transform_3 : Terminator
  Term_Carton41_Transform_2 : Terminator
  Term_Carton41_Transform_3 : Terminator
  Term_Carton42_Transform_2 : Terminator
  Term_Carton42_Transform_3 : Terminator
  Term_Carton43_Transform_2 : Terminator
  Term_Carton43_Transform_3 : Terminator
  Term_Carton44_Transform_2 : Terminator
  Term_Carton44_Transform_3 : Terminator
  Term_Carton45_Transform_2 : Terminator
  Term_Carton45_Transform_3 : Terminator
  Term_Carton46_Transform_2 : Terminator
  Term_Carton46_Transform_3 : Terminator
  Term_Carton47_Transform_2 : Terminator
  Term_Carton47_Transform_3 : Terminator
  Term_Carton48_Transform_2 : Terminator
  Term_Carton48_Transform_3 : Terminator
  Term_Carton49_Transform_2 : Terminator
  Term_Carton49_Transform_3 : Terminator
  Term_Carton50_Transform_2 : Terminator
  Term_Carton50_Transform_3 : Terminator
  Term_Carton51_Transform_2 : Terminator
  Term_Carton51_Transform_3 : Terminator
  Term_Carton52_Transform_2 : Terminator
  Term_Carton52_Transform_3 : Terminator
  Term_Carton53_Transform_2 : Terminator
  Term_Carton53_Transform_3 : Terminator
  Term_Carton54_Transform_2 : Terminator
  Term_Carton54_Transform_3 : Terminator
  Term_Phase3_Warehouse_1 : Terminator
  Trans Demux : Demux  Outputs=[3 3 3 3 3 3 3 3 3 3 3 3 3 3 3 3 3 3 3 3 3 3 3 3 3 3 3 3 3 3 3 3 3 3 3 3 3 3 3 3 3 3 3 3 3 3 3 3 3 3 3 3 3 3]
  wires:
  Carton01 Transform/1 -> Carton01 Delay/1
  Carton01 Delay/1 -> Pool Pack/1(a1)
  Carton02 Transform/1 -> Carton02 Delay/1
  Carton02 Delay/1 -> Pool Pack/2(a2)
  Carton03 Transform/1 -> Carton03 Delay/1
  Carton03 Delay/1 -> Pool Pack/3(a3)
  Carton04 Transform/1 -> Carton04 Delay/1
  Carton04 Delay/1 -> Pool Pack/4(a4)
  Carton05 Transform/1 -> Carton05 Delay/1
  Carton05 Delay/1 -> Pool Pack/5(a5)
  Carton06 Transform/1 -> Carton06 Delay/1
  Carton06 Delay/1 -> Pool Pack/6(a6)
  Carton07 Transform/1 -> Carton07 Delay/1
  Carton07 Delay/1 -> Pool Pack/7(a7)
  Carton08 Transform/1 -> Carton08 Delay/1
  Carton08 Delay/1 -> Pool Pack/8(a8)
  Carton09 Transform/1 -> Carton09 Delay/1
  Carton09 Delay/1 -> Pool Pack/9(a9)
  Carton10 Transform/1 -> Carton10 Delay/1
  Carton10 Delay/1 -> Pool Pack/10(a10)
  Carton11 Transform/1 -> Carton11 Delay/1
  Carton11 Delay/1 -> Pool Pack/11(a11)
  Carton12 Transform/1 -> Carton12 Delay/1
  Carton12 Delay/1 -> Pool Pack/12(a12)
  Carton13 Transform/1 -> Carton13 Delay/1
  Carton13 Delay/1 -> Pool Pack/13(a13)
  Carton14 Transform/1 -> Carton14 Delay/1
  Carton14 Delay/1 -> Pool Pack/14(a14)
  Carton15 Transform/1 -> Carton15 Delay/1
  Carton15 Delay/1 -> Pool Pack/15(a15)
  Carton16 Transform/1 -> Carton16 Delay/1
  Carton16 Delay/1 -> Pool Pack/16(a16)
  Carton17 Transform/1 -> Carton17 Delay/1
  Carton17 Delay/1 -> Pool Pack/17(a17)
  Carton18 Transform/1 -> Carton18 Delay/1
  Carton18 Delay/1 -> Pool Pack/18(a18)
  Carton19 Transform/1 -> Carton19 Delay/1
  Carton19 Delay/1 -> Pool Pack/19(a19)
  Carton20 Transform/1 -> Carton20 Delay/1
  Carton20 Delay/1 -> Pool Pack/20(a20)
  Carton21 Transform/1 -> Carton21 Delay/1
  Carton21 Delay/1 -> Pool Pack/21(a21)
  Carton22 Transform/1 -> Carton22 Delay/1
  Carton22 Delay/1 -> Pool Pack/22(a22)
  Carton23 Transform/1 -> Carton23 Delay/1
  Carton23 Delay/1 -> Pool Pack/23(a23)
  Carton24 Transform/1 -> Carton24 Delay/1
  Carton24 Delay/1 -> Pool Pack/24(a24)
  Carton25 Transform/1 -> Carton25 Delay/1
  Carton25 Delay/1 -> Pool Pack/25(a25)
  Carton26 Transform/1 -> Carton26 Delay/1
  Carton26 Delay/1 -> Pool Pack/26(a26)
  Carton27 Transform/1 -> Carton27 Delay/1
  Carton27 Delay/1 -> Pool Pack/27(a27)
  Carton28 Transform/1 -> Carton28 Delay/1
  Carton28 Delay/1 -> Pool Pack/28(a28)
  Carton29 Transform/1 -> Carton29 Delay/1
  Carton29 Delay/1 -> Pool Pack/29(a29)
  Carton30 Transform/1 -> Carton30 Delay/1
  Carton30 Delay/1 -> Pool Pack/30(a30)
  Carton31 Transform/1 -> Carton31 Delay/1
  Carton31 Delay/1 -> Pool Pack/31(a31)
  Carton32 Transform/1 -> Carton32 Delay/1
  Carton32 Delay/1 -> Pool Pack/32(a32)
  Carton33 Transform/1 -> Carton33 Delay/1
  Carton33 Delay/1 -> Pool Pack/33(a33)
  Carton34 Transform/1 -> Carton34 Delay/1
  Carton34 Delay/1 -> Pool Pack/34(a34)
  Carton35 Transform/1 -> Carton35 Delay/1
  Carton35 Delay/1 -> Pool Pack/35(a35)
  Carton36 Transform/1 -> Carton36 Delay/1
  Carton36 Delay/1 -> Pool Pack/36(a36)
  Carton37 Transform/1 -> Carton37 Delay/1
  Carton37 Delay/1 -> Pool Pack/37(a37)
  Carton38 Transform/1 -> Carton38 Delay/1
  Carton38 Delay/1 -> Pool Pack/38(a38)
  Carton39 Transform/1 -> Carton39 Delay/1
  Carton39 Delay/1 -> Pool Pack/39(a39)
  Carton40 Transform/1 -> Carton40 Delay/1
  Carton40 Delay/1 -> Pool Pack/40(a40)
  Carton41 Transform/1 -> Carton41 Delay/1
  Carton41 Delay/1 -> Pool Pack/41(a41)
  Carton42 Transform/1 -> Carton42 Delay/1
  Carton42 Delay/1 -> Pool Pack/42(a42)
  Carton43 Transform/1 -> Carton43 Delay/1
  Carton43 Delay/1 -> Pool Pack/43(a43)
  Carton44 Transform/1 -> Carton44 Delay/1
  Carton44 Delay/1 -> Pool Pack/44(a44)
  Carton45 Transform/1 -> Carton45 Delay/1
  Carton45 Delay/1 -> Pool Pack/45(a45)
  Carton46 Transform/1 -> Carton46 Delay/1
  Carton46 Delay/1 -> Pool Pack/46(a46)
  Carton47 Transform/1 -> Carton47 Delay/1
  Carton47 Delay/1 -> Pool Pack/47(a47)
  Carton48 Transform/1 -> Carton48 Delay/1
  Carton48 Delay/1 -> Pool Pack/48(a48)
  Carton49 Transform/1 -> Carton49 Delay/1
  Carton49 Delay/1 -> Pool Pack/49(a49)
  Carton50 Transform/1 -> Carton50 Delay/1
  Carton50 Delay/1 -> Pool Pack/50(a50)
  Carton51 Transform/1 -> Carton51 Delay/1
  Carton51 Delay/1 -> Pool Pack/51(a51)
  Carton52 Transform/1 -> Carton52 Delay/1
  Carton52 Delay/1 -> Pool Pack/52(a52)
  Carton53 Transform/1 -> Carton53 Delay/1
  Carton53 Delay/1 -> Pool Pack/53(a53)
  Carton54 Transform/1 -> Carton54 Delay/1
  Carton54 Delay/1 -> Pool Pack/54(a54)
  Pool Pack/1(y) -> Robot 5/1(Pool), Robot 6/1(Pool), Robot 4/1(Pool), Robot 3/1(Pool), Robot 2/1(Pool), Robot 1/1(Pool)
  Robot 1/1(Pose) -> Robot 1 Cam Pose/1(pose), Marker 1 Calc/1(pose), Poses Mux/1(a1), Robot 1 Sense/1
  Robot 1 Lidar Off/1 -> Robot 1 Sense/2
  Robot 1 Sense/1 -> Robot 1/2(EstPose), Robot 1 Cam Detect/3
  Robot 1 Sense/2 -> Robot 1/3(SenseBus)
  Robot 1/3(Lift) -> Robot 1 Cam Pose/2(lift), Robot 1 Cam Detect/4, Lifts Mux/1(a1)
  Robot 1 Cam Pose/1(translation) -> Robot 1 Camera/1
  Robot 1 Cam Pose/2(rotation) -> Robot 1 Camera/2
  Robot 1 Camera/1 -> Robot 1 Cam Detect/1
  Robot 1/4(State) -> Robot 1 Cam Detect/2
  Robot 1 Cam Detect/1 -> Robot 1/4(CamBus)
  Robot 2/1(Pose) -> Robot 2 Sense/1, Robot 2 Cam Pose/1(pose), Marker 2 Calc/1(pose), Poses Mux/2(a2)
  Robot 2 Lidar Off/1 -> Robot 2 Sense/2
  Robot 2 Sense/1 -> Robot 2/2(EstPose), Robot 2 Cam Detect/3
  Robot 2 Sense/2 -> Robot 2/3(SenseBus)
  Robot 2/3(Lift) -> Robot 2 Cam Pose/2(lift), Robot 2 Cam Detect/4, Lifts Mux/2(a2)
  Robot 2 Cam Pose/1(translation) -> Robot 2 Camera/1
  Robot 2 Cam Pose/2(rotation) -> Robot 2 Camera/2
  Robot 2 Camera/1 -> Robot 2 Cam Detect/1
  Robot 2/4(State) -> Robot 2 Cam Detect/2
  Robot 2 Cam Detect/1 -> Robot 2/4(CamBus)
  Robot 3/1(Pose) -> Robot 3 Sense/1, Robot 3 Cam Pose/1(pose), Marker 3 Calc/1(pose), Poses Mux/3(a3)
  Robot 3 Lidar Off/1 -> Robot 3 Sense/2
  Robot 3 Sense/1 -> Robot 3/2(EstPose), Robot 3 Cam Detect/3
  Robot 3 Sense/2 -> Robot 3/3(SenseBus)
  Robot 3/3(Lift) -> Robot 3 Cam Pose/2(lift), Robot 3 Cam Detect/4, Lifts Mux/3(a3)
  Robot 3 Cam Pose/1(translation) -> Robot 3 Camera/1
  Robot 3 Cam Pose/2(rotation) -> Robot 3 Camera/2
  Robot 3 Camera/1 -> Robot 3 Cam Detect/1
  Robot 3/4(State) -> Robot 3 Cam Detect/2
  Robot 3 Cam Detect/1 -> Robot 3/4(CamBus)
  Robot 4/1(Pose) -> Robot 4 Sense/1, Robot 4 Cam Pose/1(pose), Marker 4 Calc/1(pose), Poses Mux/4(a4)
  Robot 4 Lidar Off/1 -> Robot 4 Sense/2
  Robot 4 Sense/1 -> Robot 4/2(EstPose), Robot 4 Cam Detect/3
  Robot 4 Sense/2 -> Robot 4/3(SenseBus)
  Robot 4/3(Lift) -> Robot 4 Cam Pose/2(lift), Robot 4 Cam Detect/4, Lifts Mux/4(a4)
  Robot 4 Cam Pose/1(translation) -> Robot 4 Camera/1
  Robot 4 Cam Pose/2(rotation) -> Robot 4 Camera/2
  Robot 4 Camera/1 -> Robot 4 Cam Detect/1
  Robot 4/4(State) -> Robot 4 Cam Detect/2
  Robot 4 Cam Detect/1 -> Robot 4/4(CamBus)
  Robot 5/1(Pose) -> Robot 5 Sense/1, Robot 5 Cam Pose/1(pose), Marker 5 Calc/1(pose), Poses Mux/5(a5)
  Robot 5 Lidar Off/1 -> Robot 5 Sense/2
  Robot 5 Sense/1 -> Robot 5/2(EstPose), Robot 5 Cam Detect/3
  Robot 5 Sense/2 -> Robot 5/3(SenseBus)
  Robot 5/3(Lift) -> Robot 5 Cam Pose/2(lift), Robot 5 Cam Detect/4, Lifts Mux/5(a5)
  Robot 5 Cam Pose/1(translation) -> Robot 5 Camera/1
  Robot 5 Cam Pose/2(rotation) -> Robot 5 Camera/2
  Robot 5 Camera/1 -> Robot 5 Cam Detect/1
  Robot 5/4(State) -> Robot 5 Cam Detect/2
  Robot 5 Cam Detect/1 -> Robot 5/4(CamBus)
  Robot 6/1(Pose) -> Robot 6 Sense/1, Robot 6 Cam Pose/1(pose), Marker 6 Calc/1(pose), Poses Mux/6(a6)
  Robot 6 Lidar Off/1 -> Robot 6 Sense/2
  Robot 6 Sense/1 -> Robot 6/2(EstPose), Robot 6 Cam Detect/3
  Robot 6 Sense/2 -> Robot 6/3(SenseBus)
  Robot 6/3(Lift) -> Robot 6 Cam Pose/2(lift), Robot 6 Cam Detect/4, Lifts Mux/6(a6)
  Robot 6 Cam Pose/1(translation) -> Robot 6 Camera/1
  Robot 6 Cam Pose/2(rotation) -> Robot 6 Camera/2
  Robot 6 Camera/1 -> Robot 6 Cam Detect/1
  Robot 6/4(State) -> Robot 6 Cam Detect/2
  Robot 6 Cam Detect/1 -> Robot 6/4(CamBus)
  Robot 1/2(Pack) -> Carton Router/1(p1)
  Robot 2/2(Pack) -> Carton Router/2(p2)
  Robot 3/2(Pack) -> Carton Router/3(p3)
  Robot 4/2(Pack) -> Carton Router/4(p4)
  Robot 5/2(Pack) -> Carton Router/5(p5)
  Robot 6/2(Pack) -> Carton Router/6(p6)
  Fleet Carton Cmd/1 -> Carton Router/7(fc)
  Fleet Carton Cmd/2 -> Carton Router/8(fr)
  Fleet Carton Cmd/3 -> Carton Router/9(fa)
  Carton Router/1(trans) -> Trans Demux/1
  Carton Router/2(rot) -> Rot Demux/1
  Carton Router/3(drv) -> Drv Demux/1
  Trans Demux/1 -> Carton Driver 1/1(Translation)
  Rot Demux/1 -> Carton Driver 1/2(Rotation)
  Box Scale Hold/1 -> Marker 6a Set/3, Marker 6b Set/3, Marker 6c Set/3, Marker 4c Set/3, Marker 5a Set/3, Marker 5b Set/3, Marker 3c Set/3, Marker 4a Set/3, Marker 4b Set/3, Marker 2b Set/3, Marker 2c Set/3, Marker 3a Set/3, Marker 2a Set/3, Marker 3b Set/3, Marker 5c Set/3, Carton Driver 53/3(Scale), Carton Driver 54/3(Scale), Carton Driver 52/3(Scale), Carton Driver 51/3(Scale), Carton Driver 50/3(Scale), Carton Driver 49/3(Scale), Carton Driver 48/3(Scale), Carton Driver 47/3(Scale), Carton Driver 46/3(Scale), Carton Driver 45/3(Scale), Carton Driver 44/3(Scale), Carton Driver 43/3(Scale), Carton Driver 42/3(Scale), Carton Driver 41/3(Scale), Carton Driver 40/3(Scale), Carton Driver 39/3(Scale), Carton Driver 38/3(Scale), Carton Driver 37/3(Scale), Carton Driver 36/3(Scale), Carton Driver 35/3(Scale), Carton Driver 34/3(Scale), Carton Driver 33/3(Scale), Carton Driver 32/3(Scale), Carton Driver 31/3(Scale), Carton Driver 30/3(Scale), Carton Driver 29/3(Scale), Carton Driver 28/3(Scale), Carton Driver 27/3(Scale), Carton Driver 26/3(Scale), Carton Driver 25/3(Scale), Carton Driver 24/3(Scale), Carton Driver 23/3(Scale), Carton Driver 22/3(Scale), Carton Driver 21/3(Scale), Carton Driver 20/3(Scale), Carton Driver 19/3(Scale), Carton Driver 18/3(Scale), Carton Driver 17/3(Scale), Carton Driver 16/3(Scale), Carton Driver 15/3(Scale), Carton Driver 14/3(Scale), Carton Driver 13/3(Scale), Carton Driver 12/3(Scale), Carton Driver 11/3(Scale), Carton Driver 10/3(Scale), Carton Driver 9/3(Scale), Carton Driver 2/3(Scale), Carton Driver 3/3(Scale), Carton Driver 4/3(Scale), Carton Driver 5/3(Scale), Carton Driver 6/3(Scale), Carton Driver 7/3(Scale), Carton Driver 8/3(Scale), Carton Driver 1/3(Scale), Marker 1b Set/3, Marker 1c Set/3, Marker 1a Set/3
  Drv Demux/1 -> Carton Driver 1/Enable
  Trans Demux/2 -> Carton Driver 2/1(Translation)
  Rot Demux/2 -> Carton Driver 2/2(Rotation)
  Drv Demux/2 -> Carton Driver 2/Enable
  Trans Demux/3 -> Carton Driver 3/1(Translation)
  Rot Demux/3 -> Carton Driver 3/2(Rotation)
  Drv Demux/3 -> Carton Driver 3/Enable
  Trans Demux/4 -> Carton Driver 4/1(Translation)
  Rot Demux/4 -> Carton Driver 4/2(Rotation)
  Drv Demux/4 -> Carton Driver 4/Enable
  Trans Demux/5 -> Carton Driver 5/1(Translation)
  Rot Demux/5 -> Carton Driver 5/2(Rotation)
  Drv Demux/5 -> Carton Driver 5/Enable
  Trans Demux/6 -> Carton Driver 6/1(Translation)
  Rot Demux/6 -> Carton Driver 6/2(Rotation)
  Drv Demux/6 -> Carton Driver 6/Enable
  Trans Demux/7 -> Carton Driver 7/1(Translation)
  Rot Demux/7 -> Carton Driver 7/2(Rotation)
  Drv Demux/7 -> Carton Driver 7/Enable
  Trans Demux/8 -> Carton Driver 8/1(Translation)
  Rot Demux/8 -> Carton Driver 8/2(Rotation)
  Drv Demux/8 -> Carton Driver 8/Enable
  Trans Demux/9 -> Carton Driver 9/1(Translation)
  Rot Demux/9 -> Carton Driver 9/2(Rotation)
  Drv Demux/9 -> Carton Driver 9/Enable
  Trans Demux/10 -> Carton Driver 10/1(Translation)
  Rot Demux/10 -> Carton Driver 10/2(Rotation)
  Drv Demux/10 -> Carton Driver 10/Enable
  Trans Demux/11 -> Carton Driver 11/1(Translation)
  Rot Demux/11 -> Carton Driver 11/2(Rotation)
  Drv Demux/11 -> Carton Driver 11/Enable
  Trans Demux/12 -> Carton Driver 12/1(Translation)
  Rot Demux/12 -> Carton Driver 12/2(Rotation)
  Drv Demux/12 -> Carton Driver 12/Enable
  Trans Demux/13 -> Carton Driver 13/1(Translation)
  Rot Demux/13 -> Carton Driver 13/2(Rotation)
  Drv Demux/13 -> Carton Driver 13/Enable
  Trans Demux/14 -> Carton Driver 14/1(Translation)
  Rot Demux/14 -> Carton Driver 14/2(Rotation)
  Drv Demux/14 -> Carton Driver 14/Enable
  Trans Demux/15 -> Carton Driver 15/1(Translation)
  Rot Demux/15 -> Carton Driver 15/2(Rotation)
  Drv Demux/15 -> Carton Driver 15/Enable
  Trans Demux/16 -> Carton Driver 16/1(Translation)
  Rot Demux/16 -> Carton Driver 16/2(Rotation)
  Drv Demux/16 -> Carton Driver 16/Enable
  Trans Demux/17 -> Carton Driver 17/1(Translation)
  Rot Demux/17 -> Carton Driver 17/2(Rotation)
  Drv Demux/17 -> Carton Driver 17/Enable
  Trans Demux/18 -> Carton Driver 18/1(Translation)
  Rot Demux/18 -> Carton Driver 18/2(Rotation)
  Drv Demux/18 -> Carton Driver 18/Enable
  Trans Demux/19 -> Carton Driver 19/1(Translation)
  Rot Demux/19 -> Carton Driver 19/2(Rotation)
  Drv Demux/19 -> Carton Driver 19/Enable
  Trans Demux/20 -> Carton Driver 20/1(Translation)
  Rot Demux/20 -> Carton Driver 20/2(Rotation)
  Drv Demux/20 -> Carton Driver 20/Enable
  Trans Demux/21 -> Carton Driver 21/1(Translation)
  Rot Demux/21 -> Carton Driver 21/2(Rotation)
  Drv Demux/21 -> Carton Driver 21/Enable
  Trans Demux/22 -> Carton Driver 22/1(Translation)
  Rot Demux/22 -> Carton Driver 22/2(Rotation)
  Drv Demux/22 -> Carton Driver 22/Enable
  Trans Demux/23 -> Carton Driver 23/1(Translation)
  Rot Demux/23 -> Carton Driver 23/2(Rotation)
  Drv Demux/23 -> Carton Driver 23/Enable
  Trans Demux/24 -> Carton Driver 24/1(Translation)
  Rot Demux/24 -> Carton Driver 24/2(Rotation)
  Drv Demux/24 -> Carton Driver 24/Enable
  Trans Demux/25 -> Carton Driver 25/1(Translation)
  Rot Demux/25 -> Carton Driver 25/2(Rotation)
  Drv Demux/25 -> Carton Driver 25/Enable
  Trans Demux/26 -> Carton Driver 26/1(Translation)
  Rot Demux/26 -> Carton Driver 26/2(Rotation)
  Drv Demux/26 -> Carton Driver 26/Enable
  Trans Demux/27 -> Carton Driver 27/1(Translation)
  Rot Demux/27 -> Carton Driver 27/2(Rotation)
  Drv Demux/27 -> Carton Driver 27/Enable
  Trans Demux/28 -> Carton Driver 28/1(Translation)
  Rot Demux/28 -> Carton Driver 28/2(Rotation)
  Drv Demux/28 -> Carton Driver 28/Enable
  Trans Demux/29 -> Carton Driver 29/1(Translation)
  Rot Demux/29 -> Carton Driver 29/2(Rotation)
  Drv Demux/29 -> Carton Driver 29/Enable
  Trans Demux/30 -> Carton Driver 30/1(Translation)
  Rot Demux/30 -> Carton Driver 30/2(Rotation)
  Drv Demux/30 -> Carton Driver 30/Enable
  Trans Demux/31 -> Carton Driver 31/1(Translation)
  Rot Demux/31 -> Carton Driver 31/2(Rotation)
  Drv Demux/31 -> Carton Driver 31/Enable
  Trans Demux/32 -> Carton Driver 32/1(Translation)
  Rot Demux/32 -> Carton Driver 32/2(Rotation)
  Drv Demux/32 -> Carton Driver 32/Enable
  Trans Demux/33 -> Carton Driver 33/1(Translation)
  Rot Demux/33 -> Carton Driver 33/2(Rotation)
  Drv Demux/33 -> Carton Driver 33/Enable
  Trans Demux/34 -> Carton Driver 34/1(Translation)
  Rot Demux/34 -> Carton Driver 34/2(Rotation)
  Drv Demux/34 -> Carton Driver 34/Enable
  Trans Demux/35 -> Carton Driver 35/1(Translation)
  Rot Demux/35 -> Carton Driver 35/2(Rotation)
  Drv Demux/35 -> Carton Driver 35/Enable
  Trans Demux/36 -> Carton Driver 36/1(Translation)
  Rot Demux/36 -> Carton Driver 36/2(Rotation)
  Drv Demux/36 -> Carton Driver 36/Enable
  Trans Demux/37 -> Carton Driver 37/1(Translation)
  Rot Demux/37 -> Carton Driver 37/2(Rotation)
  Drv Demux/37 -> Carton Driver 37/Enable
  Trans Demux/38 -> Carton Driver 38/1(Translation)
  Rot Demux/38 -> Carton Driver 38/2(Rotation)
  Drv Demux/38 -> Carton Driver 38/Enable
  Trans Demux/39 -> Carton Driver 39/1(Translation)
  Rot Demux/39 -> Carton Driver 39/2(Rotation)
  Drv Demux/39 -> Carton Driver 39/Enable
  Trans Demux/40 -> Carton Driver 40/1(Translation)
  Rot Demux/40 -> Carton Driver 40/2(Rotation)
  Drv Demux/40 -> Carton Driver 40/Enable
  Trans Demux/41 -> Carton Driver 41/1(Translation)
  Rot Demux/41 -> Carton Driver 41/2(Rotation)
  Drv Demux/41 -> Carton Driver 41/Enable
  Trans Demux/42 -> Carton Driver 42/1(Translation)
  Rot Demux/42 -> Carton Driver 42/2(Rotation)
  Drv Demux/42 -> Carton Driver 42/Enable
  Trans Demux/43 -> Carton Driver 43/1(Translation)
  Rot Demux/43 -> Carton Driver 43/2(Rotation)
  Drv Demux/43 -> Carton Driver 43/Enable
  Trans Demux/44 -> Carton Driver 44/1(Translation)
  Rot Demux/44 -> Carton Driver 44/2(Rotation)
  Drv Demux/44 -> Carton Driver 44/Enable
  Trans Demux/45 -> Carton Driver 45/1(Translation)
  Rot Demux/45 -> Carton Driver 45/2(Rotation)
  Drv Demux/45 -> Carton Driver 45/Enable
  Trans Demux/46 -> Carton Driver 46/1(Translation)
  Rot Demux/46 -> Carton Driver 46/2(Rotation)
  Drv Demux/46 -> Carton Driver 46/Enable
  Trans Demux/47 -> Carton Driver 47/1(Translation)
  Rot Demux/47 -> Carton Driver 47/2(Rotation)
  Drv Demux/47 -> Carton Driver 47/Enable
  Trans Demux/48 -> Carton Driver 48/1(Translation)
  Rot Demux/48 -> Carton Driver 48/2(Rotation)
  Drv Demux/48 -> Carton Driver 48/Enable
  Trans Demux/49 -> Carton Driver 49/1(Translation)
  Rot Demux/49 -> Carton Driver 49/2(Rotation)
  Drv Demux/49 -> Carton Driver 49/Enable
  Trans Demux/50 -> Carton Driver 50/1(Translation)
  Rot Demux/50 -> Carton Driver 50/2(Rotation)
  Drv Demux/50 -> Carton Driver 50/Enable
  Trans Demux/51 -> Carton Driver 51/1(Translation)
  Rot Demux/51 -> Carton Driver 51/2(Rotation)
  Drv Demux/51 -> Carton Driver 51/Enable
  Trans Demux/52 -> Carton Driver 52/1(Translation)
  Rot Demux/52 -> Carton Driver 52/2(Rotation)
  Drv Demux/52 -> Carton Driver 52/Enable
  Trans Demux/53 -> Carton Driver 53/1(Translation)
  Rot Demux/53 -> Carton Driver 53/2(Rotation)
  Drv Demux/53 -> Carton Driver 53/Enable
  Trans Demux/54 -> Carton Driver 54/1(Translation)
  Rot Demux/54 -> Carton Driver 54/2(Rotation)
  Drv Demux/54 -> Carton Driver 54/Enable
  Marker 1 Calc/1(t1) -> Marker 1a Set/1
  Marker 1 Calc/2(r1) -> Marker 1a Set/2
  Marker 1 Calc/3(t2) -> Marker 1b Set/1
  Marker 1 Calc/4(r2) -> Marker 1b Set/2
  Marker 1 Calc/5(t3) -> Marker 1c Set/1
  Marker 1 Calc/6(r3) -> Marker 1c Set/2
  Marker 2 Calc/1(t1) -> Marker 2a Set/1
  Marker 2 Calc/2(r1) -> Marker 2a Set/2
  Marker 2 Calc/3(t2) -> Marker 2b Set/1
  Marker 2 Calc/4(r2) -> Marker 2b Set/2
  Marker 2 Calc/5(t3) -> Marker 2c Set/1
  Marker 2 Calc/6(r3) -> Marker 2c Set/2
  Marker 3 Calc/1(t1) -> Marker 3a Set/1
  Marker 3 Calc/2(r1) -> Marker 3a Set/2
  Marker 3 Calc/3(t2) -> Marker 3b Set/1
  Marker 3 Calc/4(r2) -> Marker 3b Set/2
  Marker 3 Calc/5(t3) -> Marker 3c Set/1
  Marker 3 Calc/6(r3) -> Marker 3c Set/2
  Marker 4 Calc/1(t1) -> Marker 4a Set/1
  Marker 4 Calc/2(r1) -> Marker 4a Set/2
  Marker 4 Calc/3(t2) -> Marker 4b Set/1
  Marker 4 Calc/4(r2) -> Marker 4b Set/2
  Marker 4 Calc/5(t3) -> Marker 4c Set/1
  Marker 4 Calc/6(r3) -> Marker 4c Set/2
  Marker 5 Calc/1(t1) -> Marker 5a Set/1
  Marker 5 Calc/2(r1) -> Marker 5a Set/2
  Marker 5 Calc/3(t2) -> Marker 5b Set/1
  Marker 5 Calc/4(r2) -> Marker 5b Set/2
  Marker 5 Calc/5(t3) -> Marker 5c Set/1
  Marker 5 Calc/6(r3) -> Marker 5c Set/2
  Marker 6 Calc/1(t1) -> Marker 6a Set/1
  Marker 6 Calc/2(r1) -> Marker 6a Set/2
  Marker 6 Calc/3(t2) -> Marker 6b Set/1
  Marker 6 Calc/4(r2) -> Marker 6b Set/2
  Marker 6 Calc/5(t3) -> Marker 6c Set/1
  Marker 6 Calc/6(r3) -> Marker 6c Set/2
  Poses Mux/1(y) -> Fleet Camera Pose/1(poses)
  Lifts Mux/1(y) -> Fleet Camera Pose/2(lifts)
  Fleet Camera Pose/1(translation) -> Fleet Camera/1
  Fleet Camera Pose/2(rotation) -> Fleet Camera/2
  Fleet Camera/1 -> Fleet Vision Viewer/1(img)
  Fleet Camera Pose/3(selPose) -> Fleet Vision Viewer/2(pose)
  Fleet Camera Pose/4(selLift) -> Fleet Vision Viewer/3(lift)
  Fleet Camera Pose/5(sel) -> Fleet Vision Viewer/4(sel)
  Fleet Vision Viewer/1(ok) -> Fleet Vision End/1
  Fleet Carton Cmd/4 -> Fleet Stop/1
  Carton01 Transform/2 -> Term_Carton01_Transform_2/1
  Carton01 Transform/3 -> Term_Carton01_Transform_3/1
  Carton02 Transform/2 -> Term_Carton02_Transform_2/1
  Carton02 Transform/3 -> Term_Carton02_Transform_3/1
  Carton03 Transform/2 -> Term_Carton03_Transform_2/1
  Carton03 Transform/3 -> Term_Carton03_Transform_3/1
  Carton04 Transform/2 -> Term_Carton04_Transform_2/1
  Carton04 Transform/3 -> Term_Carton04_Transform_3/1
  Carton05 Transform/2 -> Term_Carton05_Transform_2/1
  Carton05 Transform/3 -> Term_Carton05_Transform_3/1
  Carton06 Transform/2 -> Term_Carton06_Transform_2/1
  Carton06 Transform/3 -> Term_Carton06_Transform_3/1
  Carton07 Transform/2 -> Term_Carton07_Transform_2/1
  Carton07 Transform/3 -> Term_Carton07_Transform_3/1
  Carton08 Transform/2 -> Term_Carton08_Transform_2/1
  Carton08 Transform/3 -> Term_Carton08_Transform_3/1
  Carton09 Transform/2 -> Term_Carton09_Transform_2/1
  Carton09 Transform/3 -> Term_Carton09_Transform_3/1
  Carton10 Transform/2 -> Term_Carton10_Transform_2/1
  Carton10 Transform/3 -> Term_Carton10_Transform_3/1
  Carton11 Transform/2 -> Term_Carton11_Transform_2/1
  Carton11 Transform/3 -> Term_Carton11_Transform_3/1
  Carton12 Transform/2 -> Term_Carton12_Transform_2/1
  Carton12 Transform/3 -> Term_Carton12_Transform_3/1
  Carton13 Transform/2 -> Term_Carton13_Transform_2/1
  Carton13 Transform/3 -> Term_Carton13_Transform_3/1
  Carton14 Transform/2 -> Term_Carton14_Transform_2/1
  Carton14 Transform/3 -> Term_Carton14_Transform_3/1
  Carton15 Transform/2 -> Term_Carton15_Transform_2/1
  Carton15 Transform/3 -> Term_Carton15_Transform_3/1
  Carton16 Transform/2 -> Term_Carton16_Transform_2/1
  Carton16 Transform/3 -> Term_Carton16_Transform_3/1
  Carton17 Transform/2 -> Term_Carton17_Transform_2/1
  Carton17 Transform/3 -> Term_Carton17_Transform_3/1
  Carton18 Transform/2 -> Term_Carton18_Transform_2/1
  Carton18 Transform/3 -> Term_Carton18_Transform_3/1
  Carton19 Transform/2 -> Term_Carton19_Transform_2/1
  Carton19 Transform/3 -> Term_Carton19_Transform_3/1
  Carton20 Transform/2 -> Term_Carton20_Transform_2/1
  Carton20 Transform/3 -> Term_Carton20_Transform_3/1
  Carton21 Transform/2 -> Term_Carton21_Transform_2/1
  Carton21 Transform/3 -> Term_Carton21_Transform_3/1
  Carton22 Transform/2 -> Term_Carton22_Transform_2/1
  Carton22 Transform/3 -> Term_Carton22_Transform_3/1
  Carton23 Transform/2 -> Term_Carton23_Transform_2/1
  Carton23 Transform/3 -> Term_Carton23_Transform_3/1
  Carton24 Transform/2 -> Term_Carton24_Transform_2/1
  Carton24 Transform/3 -> Term_Carton24_Transform_3/1
  Carton25 Transform/2 -> Term_Carton25_Transform_2/1
  Carton25 Transform/3 -> Term_Carton25_Transform_3/1
  Carton26 Transform/2 -> Term_Carton26_Transform_2/1
  Carton26 Transform/3 -> Term_Carton26_Transform_3/1
  Carton27 Transform/2 -> Term_Carton27_Transform_2/1
  Carton27 Transform/3 -> Term_Carton27_Transform_3/1
  Carton28 Transform/2 -> Term_Carton28_Transform_2/1
  Carton28 Transform/3 -> Term_Carton28_Transform_3/1
  Carton29 Transform/2 -> Term_Carton29_Transform_2/1
  Carton29 Transform/3 -> Term_Carton29_Transform_3/1
  Carton30 Transform/2 -> Term_Carton30_Transform_2/1
  Carton30 Transform/3 -> Term_Carton30_Transform_3/1
  Carton31 Transform/2 -> Term_Carton31_Transform_2/1
  Carton31 Transform/3 -> Term_Carton31_Transform_3/1
  Carton32 Transform/2 -> Term_Carton32_Transform_2/1
  Carton32 Transform/3 -> Term_Carton32_Transform_3/1
  Carton33 Transform/2 -> Term_Carton33_Transform_2/1
  Carton33 Transform/3 -> Term_Carton33_Transform_3/1
  Carton34 Transform/2 -> Term_Carton34_Transform_2/1
  Carton34 Transform/3 -> Term_Carton34_Transform_3/1
  Carton35 Transform/2 -> Term_Carton35_Transform_2/1
  Carton35 Transform/3 -> Term_Carton35_Transform_3/1
  Carton36 Transform/2 -> Term_Carton36_Transform_2/1
  Carton36 Transform/3 -> Term_Carton36_Transform_3/1
  Carton37 Transform/2 -> Term_Carton37_Transform_2/1
  Carton37 Transform/3 -> Term_Carton37_Transform_3/1
  Carton38 Transform/2 -> Term_Carton38_Transform_2/1
  Carton38 Transform/3 -> Term_Carton38_Transform_3/1
  Carton39 Transform/2 -> Term_Carton39_Transform_2/1
  Carton39 Transform/3 -> Term_Carton39_Transform_3/1
  Carton40 Transform/2 -> Term_Carton40_Transform_2/1
  Carton40 Transform/3 -> Term_Carton40_Transform_3/1
  Carton41 Transform/2 -> Term_Carton41_Transform_2/1
  Carton41 Transform/3 -> Term_Carton41_Transform_3/1
  Carton42 Transform/2 -> Term_Carton42_Transform_2/1
  Carton42 Transform/3 -> Term_Carton42_Transform_3/1
  Carton43 Transform/2 -> Term_Carton43_Transform_2/1
  Carton43 Transform/3 -> Term_Carton43_Transform_3/1
  Carton44 Transform/2 -> Term_Carton44_Transform_2/1
  Carton44 Transform/3 -> Term_Carton44_Transform_3/1
  Carton45 Transform/2 -> Term_Carton45_Transform_2/1
  Carton45 Transform/3 -> Term_Carton45_Transform_3/1
  Carton46 Transform/2 -> Term_Carton46_Transform_2/1
  Carton46 Transform/3 -> Term_Carton46_Transform_3/1
  Carton47 Transform/2 -> Term_Carton47_Transform_2/1
  Carton47 Transform/3 -> Term_Carton47_Transform_3/1
  Carton48 Transform/2 -> Term_Carton48_Transform_2/1
  Carton48 Transform/3 -> Term_Carton48_Transform_3/1
  Carton49 Transform/2 -> Term_Carton49_Transform_2/1
  Carton49 Transform/3 -> Term_Carton49_Transform_3/1
  Carton50 Transform/2 -> Term_Carton50_Transform_2/1
  Carton50 Transform/3 -> Term_Carton50_Transform_3/1
  Carton51 Transform/2 -> Term_Carton51_Transform_2/1
  Carton51 Transform/3 -> Term_Carton51_Transform_3/1
  Carton52 Transform/2 -> Term_Carton52_Transform_2/1
  Carton52 Transform/3 -> Term_Carton52_Transform_3/1
  Carton53 Transform/2 -> Term_Carton53_Transform_2/1
  Carton53 Transform/3 -> Term_Carton53_Transform_3/1
  Carton54 Transform/2 -> Term_Carton54_Transform_2/1
  Carton54 Transform/3 -> Term_Carton54_Transform_3/1
  Phase3 Warehouse/1 -> Term_Phase3_Warehouse_1/1
